simulink model "USV_Battery_Aware_MPC_Final"  (R2025b)
settings: Solver=ode45  StartTime=0.0  StopTime=1200.0  MaxStep=0.1  RelTol=1e-3
model workspace (MAT data in the model file):
  controller_mode = 3
  initial_soc = 80
  p.usv.m = 180
  p.usv.Iz = 75
  p.usv.xg = 0.05
  p.usv.L = 2.2
  p.usv.B = 0.8
  p.usv.X_udot = -20
  p.usv.Y_vdot = -45
  p.usv.Y_rdot = -1.5
  p.usv.N_vdot = -1.5
  p.usv.N_rdot = -22
  p.usv.Xu = -25
  p.usv.Yv = -60
  p.usv.Yr = -5
  p.usv.Nv = -5
  p.usv.Nr = -30
  p.usv.Xuu = -35
  p.usv.Yvv = -120
  p.usv.Yrr = -10
  p.usv.Nvv = -10
  p.usv.Nrr = -45
  p.usv.prop.B_prop = 0.6
  p.usv.prop.arm = 0.3
  p.usv.prop.T_max_ind = 150
  p.usv.prop.T_min_ind = -50
  p.usv.prop.T_max_tot = 300
  p.usv.prop.T_min_tot = 0
  p.usv.prop.N_max = 60
  p.usv.prop.rate_max = 120
  p.usv.prop.eta_motor = 0.75
  p.usv.prop.k_loss = 0.015
  p.usv.u_max = 3
  p.usv.v_max = 1
  p.usv.r_max = 0.785398163397
  p.battery.capacity_Wh = 1200
  p.battery.capacity_J = 4320000
  p.battery.initial_soc_pct = 80
  p.battery.soc_min_pct = 5
  p.battery.soc_reserve_pct = 20
  p.battery.soc_economy_pct = 50
  p.battery.soc_max_usable = 100
  p.battery.P_hotel = 35
  p.battery.circuit.V_nominal = 24
  p.battery.circuit.V_max = 29.2
  p.battery.circuit.V_min = 20
  p.battery.circuit.R_int = 0.045
  p.battery.P_charge = 600
  p.battery.charge_efficiency = 0.92
  p.mpc.Ts = 0.25
  p.mpc.Np = 20
  p.mpc.Nc = 6
  p.mpc.weights.w_speed = 80
  p.mpc.weights.w_cte = 120
  p.mpc.weights.w_psi = 100
  p.mpc.weights.w_yaw_rate = 15
  p.mpc.weights.w_power = 0.08
  p.mpc.weights.w_rate_T = 0.05
  p.mpc.weights.w_rate_N = 0.1
  p.mpc.weights.w_soc_slack = 5000
  p.mpc.bounds.T_min = 0
  p.mpc.bounds.T_max = 300
  p.mpc.bounds.N_max = 45
  p.mpc.bounds.delta_T_max = 30
  p.mpc.bounds.delta_N_max = 12
  p.mpc.bounds.u_min = 0
  p.mpc.bounds.u_max = 2.8
  p.mpc.bounds.r_max = 0.610865238198
  p.mpc.bounds.cte_max = 10
  p.mpc.solver.max_iter = 50
  p.mpc.solver.tol = 0.0001
  p.environment.current.enabled = 1
  p.environment.current.speed = 0.35
  p.environment.current.direction = 3.14159265359
  p.environment.current.type = 'constant'
  p.environment.wind.enabled = 1
  p.environment.wind.speed = 4.5
  p.environment.wind.direction = 3.92699081699
  p.environment.wind.rho_air = 1.225
  p.environment.wind.A_frontal = 0.45
  p.environment.wind.A_lateral = 0.95
  p.environment.wind.Cd_frontal = 0.7
  p.environment.wind.Cd_lateral = 0.9
  p.environment.wave.enabled = 1
  p.environment.wave.amplitude = 15
  p.environment.wave.moment_amp = 5
  p.environment.wave.frequency = 0.8
  p.environment.wave.direction = 3.31612557879
  p.environment.wave.noise_std = 3
  p.mission.map.x_min = -200
  p.mission.map.x_max = 1600
  p.mission.map.y_min = -300
  p.mission.map.y_max = 1100
  p.mission.map.resolution = 10
  p.mission.nodes.base.id = 1
  p.mission.nodes.base.x = 0
  p.mission.nodes.base.y = 0
  p.mission.nodes.base.type = 'BASE'
  p.mission.nodes.wp1.id = 2
  p.mission.nodes.wp1.x = 350
  p.mission.nodes.wp1.y = 250
  p.mission.nodes.wp1.type = 'WAYPOINT'
  p.mission.nodes.wp2.id = 3
  p.mission.nodes.wp2.x = 750
  p.mission.nodes.wp2.y = 450
  p.mission.nodes.wp2.type = 'WAYPOINT'
  p.mission.nodes.dock.id = 4
  p.mission.nodes.dock.x = 600
  p.mission.nodes.dock.y = 150
  p.mission.nodes.dock.type = 'CHARGING_DOCK'
  p.mission.nodes.harbor.id = 5
  p.mission.nodes.harbor.x = 200
  p.mission.nodes.harbor.y = 600
  p.mission.nodes.harbor.type = 'SAFE_HARBOR'
  p.mission.nodes.dest.id = 6
  p.mission.nodes.dest.x = 1200
  p.mission.nodes.dest.y = 650
  p.mission.nodes.dest.type = 'DESTINATION'
  p.mission.obstacles(1).type = 'circle'
  p.mission.obstacles(1).center = [500 380]
  p.mission.obstacles(1).radius = 90
  p.mission.obstacles(1).vertices = []
  p.mission.obstacles(2).type = 'polygon'
  p.mission.obstacles(2).center = []
  p.mission.obstacles(2).radius = []
  p.mission.obstacles(2).vertices = [850  200; 1050  250; 1000  450; 800  380]
  p.mission.obstacles(3).type = 'circle'
  p.mission.obstacles(3).center = [250 -100]
  p.mission.obstacles(3).radius = 70
  p.mission.obstacles(3).vertices = []
  p.mission.route.weights.w_distance = 0.35
  p.mission.route.weights.w_energy = 0.45
  p.mission.route.weights.w_time = 0.15
  p.mission.route.weights.w_risk = 0.05
  p.mission.guidance.R_capture_wp = 15
  p.mission.guidance.R_capture_dest = 8
  p.mission.guidance.Delta_LOS = 25
  p.mission.speeds.u_nominal = 2
  p.mission.speeds.u_economy = 1.4
  p.mission.speeds.u_low_power = 0.9
  p.mission.speeds.u_docking = 0.4
  p.mission.safety_margin = 0.25
  plan_mode = 2
settings Model: Creator=kiran  LastModifiedBy=kiran

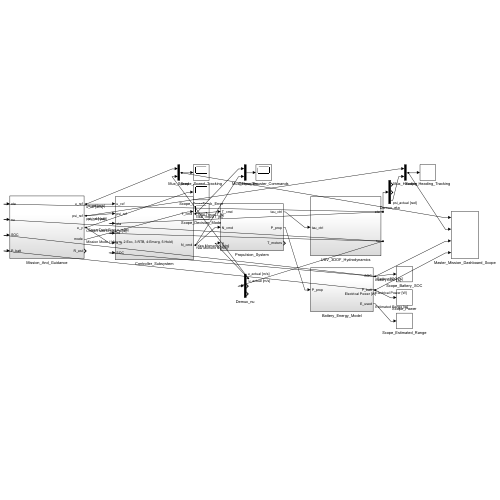
[thumbnail: Simulink's stored preview of the top-level diagram]
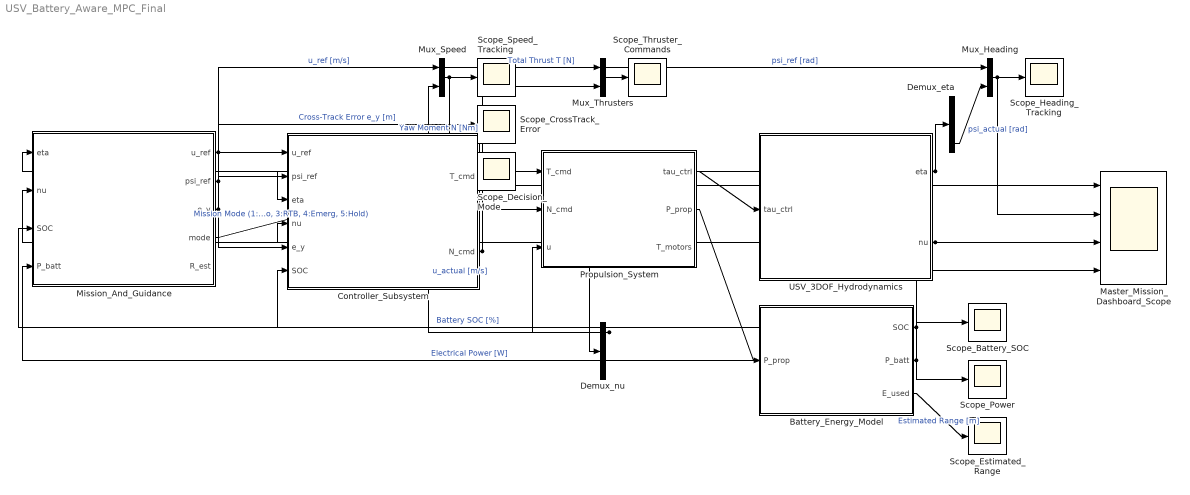
== system USV_Battery_Aware_MPC_Final ==
  Battery_Energy_Model : Subsystem
  Controller_Subsystem : Subsystem
  Demux_eta : Demux  Outputs=3
  Demux_nu : Demux  Outputs=3
  Master_Mission_Dashboard_Scope : Scope  NumInputPorts=4
      settings: ActiveDisplayString=4  Title=Total Power [W]
  Mission_And_Guidance : Subsystem
  Mux_Heading : Mux  Inputs=2
  Mux_Speed : Mux  Inputs=2
  Mux_Thrusters : Mux  Inputs=2
  Propulsion_System : Subsystem
  Scope_Battery_SOC : Scope
      settings: Title=Battery State of Charge (SOC)  YLabel=SOC [%]
  Scope_CrossTrack_Error : Scope
      settings: Title=Cross-Track Path Error (LOS Guidance)  YLabel=Cross-Track Error [m]
  Scope_Decision_Mode : Scope
      settings: Title=Battery-Aware Mission Decision Mode  YLabel=Mode State
  Scope_Estimated_Range : Scope
      settings: Title=Estimated Achievable Range at Current Speed  YLabel=Range [m]
  Scope_Heading_Tracking : Scope
      settings: Title=USV Heading Tracking: Target vs Actual  YLabel=Heading [rad]
  Scope_Power : Scope
      settings: Title=Total Electrical Power Draw  YLabel=Power [W]
  Scope_Speed_Tracking : Scope
      settings: Title=USV Surge Speed Tracking: Target vs Measured  YLabel=Speed [m/s]
  Scope_Thruster_Commands : Scope
      settings: Title=Propulsion Actuation Commands (Thrust & Moment)  YLabel=Actuation Command
  USV_3DOF_Hydrodynamics : Subsystem
  wires:
  USV_3DOF_Hydrodynamics/1(eta) -> Mission_And_Guidance/1(eta), Controller_Subsystem/3(eta), Demux_eta/1
  USV_3DOF_Hydrodynamics/2(nu) -> Mission_And_Guidance/2(nu), Controller_Subsystem/4(nu), Demux_nu/1
  Battery_Energy_Model/1(SOC) -> Mission_And_Guidance/3(SOC), Controller_Subsystem/6(SOC), Scope_Battery_SOC/1, Master_Mission_Dashboard_Scope/3  "Battery SOC [%]"
  Battery_Energy_Model/2(P_batt) -> Mission_And_Guidance/4(P_batt), Scope_Power/1, Master_Mission_Dashboard_Scope/4  "Electrical Power [W]"
  Mission_And_Guidance/1(u_ref) -> Controller_Subsystem/1(u_ref), Mux_Speed/1  "u_ref [m/s]"
  Mission_And_Guidance/2(psi_ref) -> Controller_Subsystem/2(psi_ref), Mux_Heading/1  "psi_ref [rad]"
  Mission_And_Guidance/3(e_y) -> Controller_Subsystem/5(e_y), Scope_CrossTrack_Error/1  "Cross-Track Error e_y [m]"
  Controller_Subsystem/1(T_cmd) -> Propulsion_System/1(T_cmd), Mux_Thrusters/1  "Total Thrust T [N]"
  Controller_Subsystem/2(N_cmd) -> Propulsion_System/2(N_cmd), Mux_Thrusters/2  "Yaw Moment N [Nm]"
  Demux_nu/1 -> Propulsion_System/3(u), Mux_Speed/2  "u_actual [m/s]"
  Propulsion_System/1(tau_ctrl) -> USV_3DOF_Hydrodynamics/1(tau_ctrl)
  Propulsion_System/2(P_prop) -> Battery_Energy_Model/1(P_prop)
  Mux_Speed/1 -> Scope_Speed_Tracking/1, Master_Mission_Dashboard_Scope/1
  Demux_eta/3 -> Mux_Heading/2  "psi_actual [rad]"
  Mux_Heading/1 -> Scope_Heading_Tracking/1, Master_Mission_Dashboard_Scope/2
  Mux_Thrusters/1 -> Scope_Thruster_Commands/1
  Battery_Energy_Model/3(E_used) -> Scope_Estimated_Range/1  "Estimated Range [m]"
  Mission_And_Guidance/4(mode) -> Scope_Decision_Mode/1  "Mission Mode (1:Norm, 2:Eco, 3:RTB, 4:Emerg, 5:Hold)"

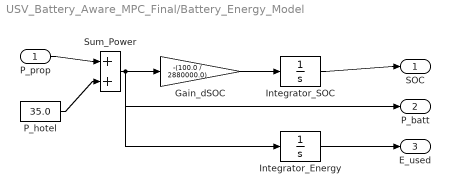
== system USV_Battery_Aware_MPC_Final/Battery_Energy_Model ==
  P_prop : Inport
  Gain_dSOC : Gain  Gain=-(100.0 / 2880000.0)
  Integrator_Energy : Integrator  InitialCondition=0.0
  Integrator_SOC : Integrator  InitialCondition=80.0  LimitOutput=on  UpperSaturationLimit=100.0  LowerSaturationLimit=0.0
  P_hotel : Constant  Value=35.0
  Sum_Power : Sum
  SOC : Outport
  P_batt : Outport  Port=2
  E_used : Outport  Port=3
  wires:
  P_prop/1 -> Sum_Power/1
  P_hotel/1 -> Sum_Power/2
  Sum_Power/1 -> Gain_dSOC/1, Integrator_Energy/1, P_batt/1
  Gain_dSOC/1 -> Integrator_SOC/1
  Integrator_SOC/1 -> SOC/1
  Integrator_Energy/1 -> E_used/1

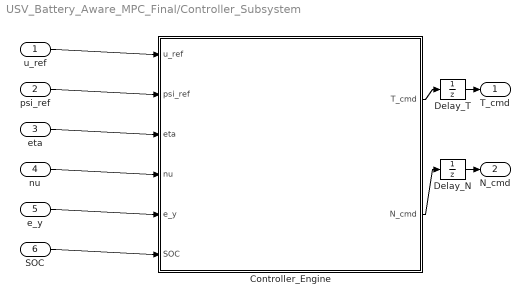
== system USV_Battery_Aware_MPC_Final/Controller_Subsystem ==
  u_ref : Inport
  psi_ref : Inport  Port=2
  eta : Inport  Port=3
  nu : Inport  Port=4
  e_y : Inport  Port=5
  SOC : Inport  Port=6
  Controller_Engine : MATLAB Function  TreatAsAtomicUnit=on
  Delay_N : UnitDelay  SampleTime=0.1  HasFrameUpgradeWarning=on
  Delay_T : UnitDelay  SampleTime=0.1  HasFrameUpgradeWarning=on
  T_cmd : Outport
  N_cmd : Outport  Port=2
  wires:
  u_ref/1 -> Controller_Engine/1(u_ref)
  psi_ref/1 -> Controller_Engine/2(psi_ref)
  eta/1 -> Controller_Engine/3(eta)
  nu/1 -> Controller_Engine/4(nu)
  e_y/1 -> Controller_Engine/5(e_y)
  SOC/1 -> Controller_Engine/6(SOC)
  Controller_Engine/1(T_cmd) -> Delay_T/1
  Controller_Engine/2(N_cmd) -> Delay_N/1
  Delay_T/1 -> T_cmd/1
  Delay_N/1 -> N_cmd/1

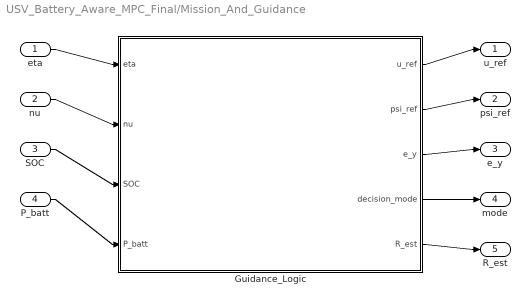
== system USV_Battery_Aware_MPC_Final/Mission_And_Guidance ==
  eta : Inport
  nu : Inport  Port=2
  SOC : Inport  Port=3
  P_batt : Inport  Port=4
  Guidance_Logic : MATLAB Function  TreatAsAtomicUnit=on
  u_ref : Outport
  psi_ref : Outport  Port=2
  e_y : Outport  Port=3
  mode : Outport  Port=4
  R_est : Outport  Port=5
  wires:
  eta/1 -> Guidance_Logic/1(eta)
  nu/1 -> Guidance_Logic/2(nu)
  SOC/1 -> Guidance_Logic/3(SOC)
  P_batt/1 -> Guidance_Logic/4(P_batt)
  Guidance_Logic/1(u_ref) -> u_ref/1
  Guidance_Logic/2(psi_ref) -> psi_ref/1
  Guidance_Logic/3(e_y) -> e_y/1
  Guidance_Logic/4(decision_mode) -> mode/1
  Guidance_Logic/5(R_est) -> R_est/1

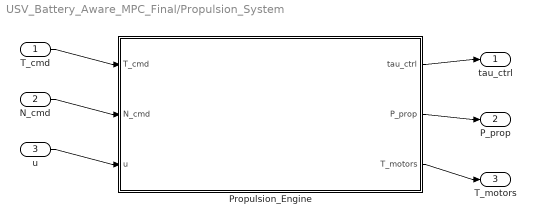
== system USV_Battery_Aware_MPC_Final/Propulsion_System ==
  T_cmd : Inport
  N_cmd : Inport  Port=2
  u : Inport  Port=3
  Propulsion_Engine : MATLAB Function  TreatAsAtomicUnit=on
  tau_ctrl : Outport
  P_prop : Outport  Port=2
  T_motors : Outport  Port=3
  wires:
  T_cmd/1 -> Propulsion_Engine/1(T_cmd)
  N_cmd/1 -> Propulsion_Engine/2(N_cmd)
  u/1 -> Propulsion_Engine/3(u)
  Propulsion_Engine/1(tau_ctrl) -> tau_ctrl/1
  Propulsion_Engine/2(P_prop) -> P_prop/1
  Propulsion_Engine/3(T_motors) -> T_motors/1

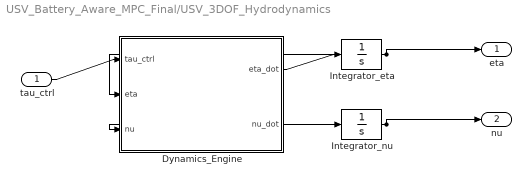
== system USV_Battery_Aware_MPC_Final/USV_3DOF_Hydrodynamics ==
  tau_ctrl : Inport
  Dynamics_Engine : MATLAB Function  TreatAsAtomicUnit=on
  Integrator_eta : Integrator  InitialCondition=[0; 0; 0]
  Integrator_nu : Integrator  InitialCondition=[0; 0; 0]
  eta : Outport
  nu : Outport  Port=2
  wires:
  tau_ctrl/1 -> Dynamics_Engine/1(tau_ctrl)
  Integrator_eta/1 -> Dynamics_Engine/2(eta), eta/1
  Integrator_nu/1 -> Dynamics_Engine/3(nu), nu/1
  Dynamics_Engine/1(eta_dot) -> Integrator_eta/1
  Dynamics_Engine/2(nu_dot) -> Integrator_nu/1

== matlab function USV_Battery_Aware_MPC_Final/Controller_Subsystem/Controller_Engine ==
  data: u_ref input; T_cmd output; psi_ref input; eta input; nu input; e_y input; SOC input; N_cmd output
function [T_cmd, N_cmd] = Controller_Engine(u_ref, psi_ref, eta, nu, e_y, SOC)
u = nu(1);
e_u = u_ref - u;
k_p_u = 220.0;
k_d_u = 45.0;
if SOC < 30.0
    k_p_u = 160.0;
end
T_raw = k_p_u * e_u - k_d_u * u;
T_cmd = min(max(T_raw, -300.0), 400.0);
psi = eta(3);
r = nu(3);
e_psi = atan2(sin(psi_ref - psi), cos(psi_ref - psi));
k_p_psi = 180.0;
k_d_psi = 55.0;
k_ey    = 15.0;
N_raw = k_p_psi * e_psi - k_d_psi * r + k_ey * e_y;
N_cmd = min(max(N_raw, -150.0), 150.0);
end

== matlab function USV_Battery_Aware_MPC_Final/Mission_And_Guidance/Guidance_Logic ==
  data: eta input; u_ref output; nu input; SOC input; P_batt input; psi_ref output; e_y output; decision_mode output; R_est output
function [u_ref, psi_ref, e_y, decision_mode, R_est] = Guidance_Logic(eta, nu, SOC, P_batt)
waypoints = [  0,   0;
             200, 150;
             500, 350;
             800, 350;
            1000, 600;
            1200, 800];
x = eta(1); y = eta(2); psi = eta(3); u = nu(1);
dists = (waypoints(:,1) - x).^2 + (waypoints(:,2) - y).^2;
min_idx = 1; min_d = dists(1);
for k = 2:6
    if dists(k) < min_d
        min_d = dists(k);
        min_idx = k;
    end
end
wp_idx = min(max(min_idx + 1, 2), 6);
curr_wp = waypoints(wp_idx, :);
prev_wp = waypoints(wp_idx - 1, :);
dx = curr_wp(1) - prev_wp(1);
dy = curr_wp(2) - prev_wp(2);
path_angle = atan2(dy, dx);
e_y = -(x - prev_wp(1))*sin(path_angle) + (y - prev_wp(2))*cos(path_angle);
Delta = 40.0;
psi_ref = path_angle - atan2(e_y, Delta);
if SOC > 40.0
    decision_mode = 1.0;
    u_ref = 2.0;
elseif SOC > 20.0
    decision_mode = 2.0;
    u_ref = 1.2;
else
    decision_mode = 3.0;
    u_ref = 0.9;
end
P_tot = max(P_batt, 40.0);
E_rem = (SOC / 100.0) * 2880000.0;
R_est = (E_rem / P_tot) * max(u, 0.8);
end

== matlab function USV_Battery_Aware_MPC_Final/Propulsion_System/Propulsion_Engine ==
  data: T_cmd input; N_cmd input; u input; tau_ctrl output; P_prop output; T_motors output
function [tau_ctrl, P_prop, T_motors] = Propulsion_Engine(T_cmd, N_cmd, u)
B = 0.54;
T_L = min(max(0.5 * T_cmd - (N_cmd / B), -400.0), 400.0);
T_R = min(max(0.5 * T_cmd + (N_cmd / B), -400.0), 400.0);
tau_ctrl = [T_L + T_R; 0.0; (T_R - T_L) * (B / 2.0)];
T_motors = [T_L; T_R];
eta_m = 0.72;
c_prop = 12.5;
u_adv = max(u, 0.1);
P_hyd_L = abs(T_L) * (u_adv + c_prop * sqrt(max(abs(T_L), 0.0)));
P_hyd_R = abs(T_R) * (u_adv + c_prop * sqrt(max(abs(T_R), 0.0)));
P_prop = (P_hyd_L + P_hyd_R) / eta_m;
end

== matlab function USV_Battery_Aware_MPC_Final/USV_3DOF_Hydrodynamics/Dynamics_Engine ==
  data: tau_ctrl input; eta_dot output; eta input; nu input; nu_dot output
function [eta_dot, nu_dot] = Dynamics_Engine(tau_ctrl, eta, nu)
psi = eta(3);
u = nu(1); v = nu(2); r = nu(3);
R = [cos(psi), -sin(psi), 0;
     sin(psi),  cos(psi), 0;
     0,         0,        1];
eta_dot = R * nu;
m11 = 205.0; m22 = 245.0; m33 = 150.0;
c13 = -m22 * v; c23 = m11 * u;
d11 = 25.0 * u + 40.0 * abs(u) * u;
d22 = 50.0 * v + 70.0 * abs(v) * v;
d33 = 35.0 * r + 45.0 * abs(r) * r;
tau_env = [8.0 * cos(0.01*eta(1)); -12.0 * sin(0.01*eta(2)); 4.0 * cos(0.05*psi)];
F_u = tau_ctrl(1) + tau_env(1) - c13*r - d11;
F_v = tau_ctrl(2) + tau_env(2) - c23*r - d22;
F_r = tau_ctrl(3) + tau_env(3) - (c23*v - c13*u) - d33;
nu_dot = [F_u / m11; F_v / m22; F_r / m33];
end
